simulink model "Controlador"  (R2023b)
settings: Solver=VariableStepAuto  StartTime=0.0  StopTime=10.0  RelTol=1e-3
values from neighbouring files (symbols this model uses):
  Bm = 0.00236    [Parametros.m]
  Jm = 0.0001    [Parametros.m]
  Kt = 0.214669    [Parametros.m]
  La = 6    [Parametros.m]
  Ra = 1.5    [Parametros.m]
  Tl = 0.40825    [Parametros.m]
libraries: simulink x1, SignalEditorBlockLib x1
settings Model: Creator=bruno  LastModifiedBy=bruno

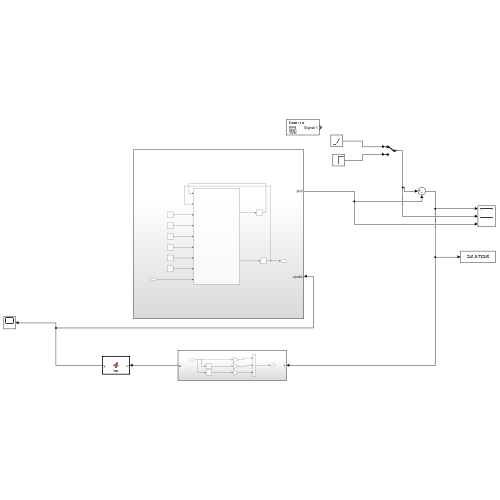
[thumbnail: Simulink's stored preview of the top-level diagram]
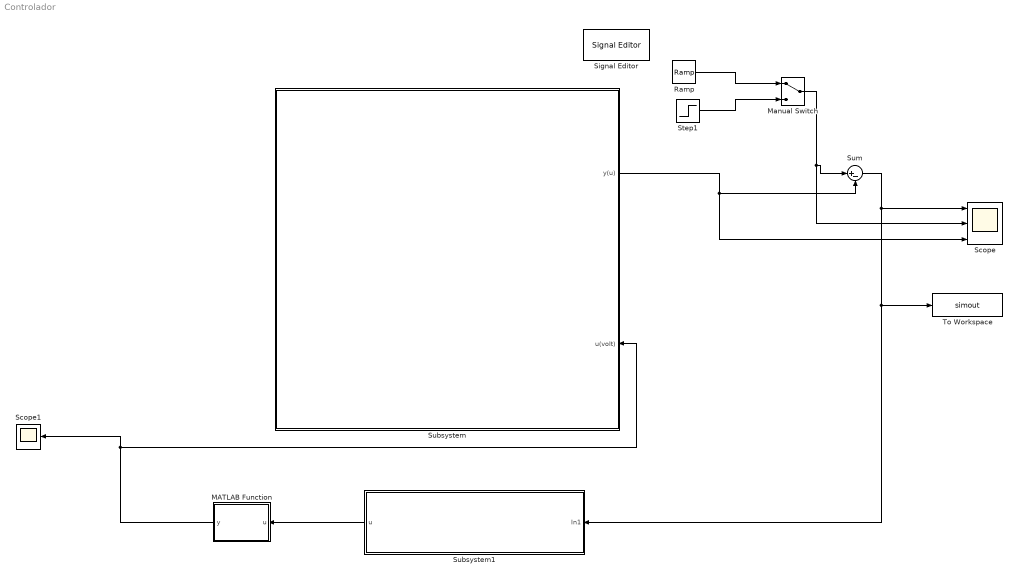
== system Controlador ==
  MATLAB Function : MATLAB Function  TreatAsAtomicUnit=on
  Manual Switch : ManualSwitch
  Ramp : simulink/Sources/Ramp  slope=1  start=0  InitialOutput=0
  Scope : Scope  NumInputPorts=3
  Scope1 : Scope
  Signal Editor : SignalEditorBlockLib/Signal Editor  FileName=untitled.mat  ActiveScenario=Scenario  ActiveSignal=Signal 1  IsBus=off  OutputBusObjectStr=Bus: BusObject  SampleTime=0  Interpolate=off  ZeroCross=off  OutputAfterFinalValue=Setting to zero  Unit=inherit  PreserveSignalName=on  ApplySigPropsToAllScenarios=on  ApplySigPropsToAllSignals=off
  Step1 : Step  SampleTime=0
  Subsystem : Subsystem
      settings: PortSchema="{\"entries\":[{\"content\":{\"sides\":[{\"content\":{},\"type\":\"ConnectorPlacement.EquallySpacedRectSide\",\"uuid\":\"4daf2f7b-7384-4cdb-89e7-add9135f52ef\"},{\"content\":{\"connectorIds\":[\"Out1\",\"In1\"],\"side\":\"RIGHT\"},\"type\":\"ConnectorPlacement.EquallySpacedRectSide\",\"uuid\":\"8719a40a-08f8-4892-81f1-ce6eb0ef35af\"},{\"content\":{\"side\":\"TOP\"},\"type\":\"ConnectorPlacement.EquallySpacedRectSide\",\"uuid\":\"bec4af6f-d1e4-4005-8ce8-d33a94b757c6\"}]},\"type\":\"ConnectorPlacement.EquallySpacedConnector\",\"uuid\":\"e20dfc7d-536d-4512-bbbd-e87edc8af37b\"}],\"packageUris\":[\"http://schema.mathworks.com/mf0/Connector/R2020b\"],\"version\":\"1.0\"}"
  Subsystem1 : Subsystem
      settings: PortSchema="{\"entries\":[{\"content\":{\"sides\":[{\"content\":{\"connectorIds\":[\"Out1\"]},\"type\":\"ConnectorPlacement.EquallySpacedRectSide\",\"uuid\":\"4daf2f7b-7384-4cdb-89e7-add9135f52ef\"},{\"content\":{\"connectorIds\":[\"In1\"],\"side\":\"RIGHT\"},\"type\":\"ConnectorPlacement.EquallySpacedRectSide\",\"uuid\":\"8719a40a-08f8-4892-81f1-ce6eb0ef35af\"},{\"content\":{\"side\":\"TOP\"},\"type\":\"ConnectorPlacement.EquallySpacedRectSide\",\"uuid\":\"bec4af6f-d1e4-4005-8ce8-d33a94b757c6\"}]},\"type\":\"ConnectorPlacement.EquallySpacedConnector\",\"uuid\":\"e20dfc7d-536d-4512-bbbd-e87edc8af37b\"}],\"packageUris\":[\"http://schema.mathworks.com/mf0/Connector/R2020b\"],\"version\":\"1.0\"}"
  Sum : Sum  Inputs=|+-
  To Workspace : ToWorkspace  VariableName=simout  SaveFormat=Timeseries  SampleTime=-1
  wires:
  MATLAB Function/1(y) -> Scope1/1, Subsystem/1(u(volt))
  Ramp/1 -> Manual Switch/1
  Step1/1 -> Manual Switch/2
  Manual Switch/1 -> Scope/2, Sum/1
  Subsystem/1(y(u)) -> Sum/2, Scope/3
  Sum/1 -> Scope/1, To Workspace/1, Subsystem1/1(In1)
  Subsystem1/1(u) -> MATLAB Function/1(u)

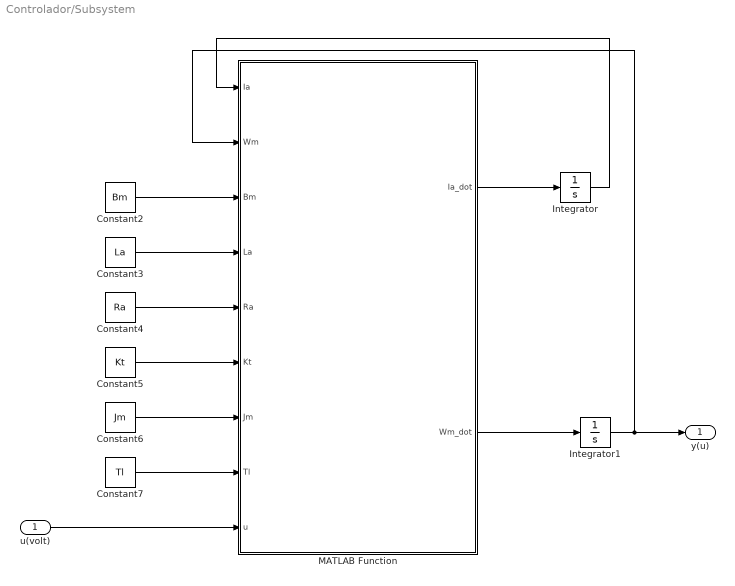
== system Controlador/Subsystem ==
  u(volt) : Inport
  Constant2 : Constant  Value=Bm
  Constant3 : Constant  Value=La
  Constant4 : Constant  Value=Ra
  Constant5 : Constant  Value=Kt
  Constant6 : Constant  Value=Jm
  Constant7 : Constant  Value=Tl
  Integrator : Integrator
  Integrator1 : Integrator
  MATLAB Function : MATLAB Function  TreatAsAtomicUnit=on
  y(u) : Outport
  wires:
  u(volt)/1 -> MATLAB Function/9(u)
  Integrator/1 -> MATLAB Function/1(Ia)
  Integrator1/1 -> y(u)/1, MATLAB Function/2(Wm)
  Constant2/1 -> MATLAB Function/3(Bm)
  Constant3/1 -> MATLAB Function/4(La)
  Constant4/1 -> MATLAB Function/5(Ra)
  Constant5/1 -> MATLAB Function/6(Kt)
  Constant6/1 -> MATLAB Function/7(Jm)
  Constant7/1 -> MATLAB Function/8(Tl)
  MATLAB Function/1(Ia_dot) -> Integrator/1
  MATLAB Function/2(Wm_dot) -> Integrator1/1

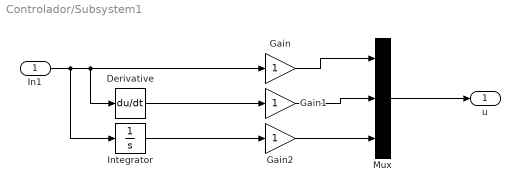
== system Controlador/Subsystem1 ==
  In1 : Inport
  Derivative : Derivative
  Gain : Gain
  Gain1 : Gain
  Gain2 : Gain
  Integrator : Integrator
  Mux : Mux  Inputs=3
  u : Outport
  wires:
  Derivative/1 -> Gain1/1
  Integrator/1 -> Gain2/1
  In1/1 -> Integrator/1, Derivative/1, Gain/1
  Gain/1 -> Mux/1
  Gain1/1 -> Mux/2
  Gain2/1 -> Mux/3
  Mux/1 -> u/1

== matlab function Controlador/MATLAB Function ==
  data: u input; y output
function y = fcn(u)

if u>=12
y = 12;

elseif u<=-12
    y=-12;

else
    y = u;
end
end

== matlab function Controlador/Subsystem/MATLAB Function ==
  data: Ia input; Wm input; Bm input; La input; Ra input; Kt input; Jm input; Tl input; u input; Ia_dot output; Wm_dot output
function [Ia_dot,Wm_dot] = fcn (Ia, Wm, Bm, La, Ra, Kt, Jm, Tl, u)

    Ia_dot= -(Ra/La)*Ia-(Kt/La)*Wm(1/La)*u;
    Wm_dot=(Kt/Jm)*Ia-(Bm/Jm)*Wm-(1/Jm)*Tl;
end
